simulink model "Mdl_BianchiOL_BladeB_WindFiltered"  (R2023a)
settings: Solver=FixedStepAuto  StartTime=0.0  StopTime=10.0  FixedStep=DT  RelTol=1e-3
values from neighbouring files (symbols this model uses):
  beta = 0.0 0.0017453292519943296 0.0034906585039886592 0.005235987755982989 0.0069813170079773184 0.0087266462599716477 0.010471975511965978 0.012217304763960306 0.013962634015954637 0.015707963267948967 0.017453292519943295 0.019198621771937627 0.020943951023931956 0.022689280275926284 0.024434609527920613 0.026179938779914941 0.027925268031909273 0.029670597283903605 0.031415926535897934 0.033161255787    [DD_Mdl1.sldd]
  Cq = 0.0 0.0 0.0 0.0 0.0 0.0 0.0 0.0 0.0 0.0 0.0 0.0 0.0 0.0 0.0 0.0 0.0 0.0 0.0 0.0 0.0 0.0 0.0 0.0 0.0 0.0 0.0 0.0 0.0 0.0 0.0 0.0 0.0 0.0 0.0 0.0 0.0 0.0 0.0 0.0 0.0 0.0 0.0 0.0 0.0 0.0 0.0 0.0 0.0 0.0 0.0 0.0 0.0 0.0 0.0 0.0 0.0 0.0 0.0 0.0 0.0 0.0 0.0 0.0 0.0 0.0 0.0 0.0 0.0 0.0 0.0 0.0 0.0 0.0 0.0 0.0 0.0 0.0 0.0 0.0 0.0 0.0 0.0 0.0 0.0 0.0 0.0 0.0 0.0 0.0 0.0 0.0 0.0 0.0 0.0 0.0 0.0 0.0 0.0 0.0    [DD_Mdl1.sldd]
  Ct = 0.0 0.0 0.0 0.0 0.0 0.0 0.0 0.0 0.0 0.0 0.0 0.0 0.0 0.0 0.0 0.0 0.0 0.0 0.0 0.0 0.0 0.0 0.0 0.0 0.0 0.0 0.0 0.0 0.0 0.0 0.0 0.0 0.0 0.0 0.0 0.0 0.0 0.0 0.0 0.0 0.0 0.0 0.0 0.0 0.0 0.0 0.0 0.0 0.0 0.0 0.0 0.0 0.0 0.0 0.0 0.0 0.0 0.0 0.0 0.0 0.0 0.0 0.0 0.0 0.0 0.0 0.0 0.0 0.0 0.0 0.0 0.0 0.0 0.0 0.0 0.0 0.0 0.0 0.0 0.0 0.0 0.0 0.0 0.0 0.0 0.0 0.0 0.0 0.0 0.0 0.0 0.0 0.0 0.0 0.0 0.0 0.0 0.0 0.0 0.0    [DD_Mdl1.sldd]
  lambda = 0.0 0.1 0.2 0.30000000000000004 0.4 0.5 0.60000000000000009 0.70000000000000007 0.8 0.9 1.0 1.1 1.2000000000000002 1.3 1.4000000000000001 1.5 1.6 1.7000000000000002 1.8 1.9000000000000001 2.0 2.1 2.2 2.3000000000000003 2.4000000000000004 2.5 2.6 2.7 2.8000000000000003 2.9000000000000004 3.0 3.1 3.2 3.3000000000000003 3.4000000000000004 3.5 3.6 3.7 3.8000000000000003 3.9000000000000004 4.0 4.100000    [DD_Mdl1.sldd]
  rho = 1.225    [DD_Mdl1.sldd]
  wecs = 3.0    [DD_Mdl1.sldd]    (also in wecsmatfile.m = struct)
libraries: Lib_WindFilter x1
Description:
  | Mdl2 (Mdl_BianchiOL_WindFiltered) with the blade model variant B (getBladeModelVersion B1/B2): WECS/BladeSchedule (bladeParamsMdl2) and WECS/LagrangeDyn instead of the constant matrix gains M\Q, M\K5, M\Ce
settings Model: DataDictionary=DD_Mdl1.sldd  Creator=ditt_aj  LastModifiedBy=jdi
settings SolverCC: AlgebraicLoopSolver=TrustRegion
settings DebuggingCC: UnconnectedInputMsg=warning  UnconnectedOutputMsg=warning  UnconnectedLineMsg=warning
settings ModelReferenceCC: EnableRefExpFcnMdlSchedulingChecks=on
settings SFSimCC: CustomCodeUndefinedFunction=UseInterfaceOnly
settings RTWCC: DLArmComputeVersion=19.05

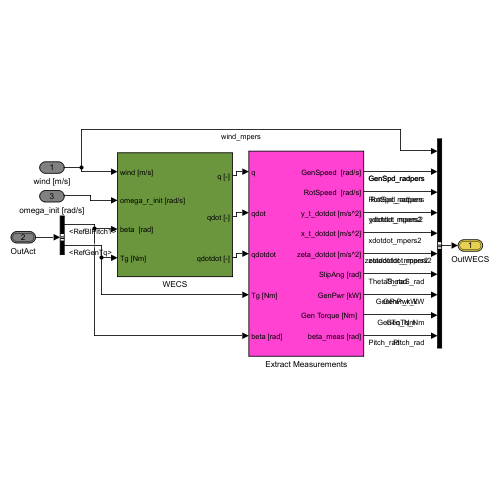
[thumbnail: Simulink's stored preview of the top-level diagram]
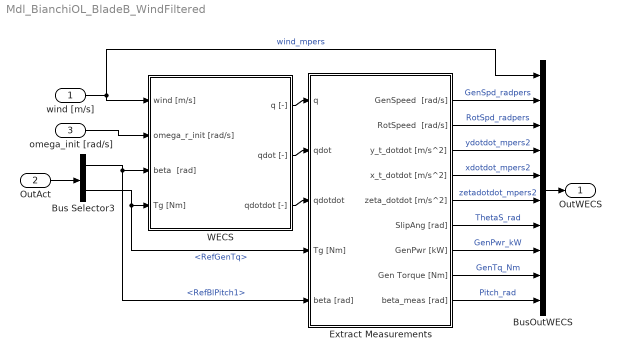
== system Mdl_BianchiOL_BladeB_WindFiltered ==
  wind [m/s] : Inport
  OutAct : Inport  Port=2  OutDataTypeStr=Bus: slBus2
  omega_init [rad/s] : Inport  Port=3
  Bus Selector3 : BusSelector  OutputSignals=RefBlPitch1,RefGenTq
  BusOutWECS : BusCreator  Inputs=10  OutDataTypeStr=Bus: slBus1
  Extract Measurements : Subsystem
  WECS : Subsystem
  OutWECS : Outport  OutDataTypeStr=Bus: slBus1
  wires:
  WECS/3(qdotdot [-]) -> Extract Measurements/3(qdotdot)
  omega_init [rad/s]/1 -> WECS/2(omega_r_init [rad/s])
  WECS/2(qdot [-]) -> Extract Measurements/2(qdot)
  WECS/1(q [-]) -> Extract Measurements/1(q)
  Extract Measurements/7(GenPwr [kW]) -> BusOutWECS/8  "GenPwr_kW"
  Extract Measurements/4(x_t_dotdot [m/s^2]) -> BusOutWECS/5  "xdotdot_mpers2"
  Extract Measurements/5(zeta_dotdot [m/s^2]) -> BusOutWECS/6  "zetadotdot_mpers2"
  Extract Measurements/6(SlipAng [rad]) -> BusOutWECS/7  "ThetaS_rad"
  Extract Measurements/9(beta_meas [rad]) -> BusOutWECS/10  "Pitch_rad"
  Extract Measurements/8("Gen Torque [Nm]  ") -> BusOutWECS/9  "GenTq_Nm"
  Extract Measurements/2(RotSpeed  [rad/s]) -> BusOutWECS/3  "RotSpd_radpers"
  Extract Measurements/3(y_t_dotdot [m/s^2]) -> BusOutWECS/4  "ydotdot_mpers2"
  BusOutWECS/1 -> OutWECS/1
  wind [m/s]/1 -> BusOutWECS/1, WECS/1(wind [m/s])  "wind_mpers"
  Extract Measurements/1(GenSpeed  [rad/s]) -> BusOutWECS/2  "GenSpd_radpers"
  OutAct/1 -> Bus Selector3/1
  Bus Selector3/2 -> Extract Measurements/4(Tg [Nm]), WECS/4(Tg [Nm])  "<RefGenTq>"
  Bus Selector3/1 -> Extract Measurements/5(beta [rad]), WECS/3(beta  [rad])  "<RefBlPitch1>"

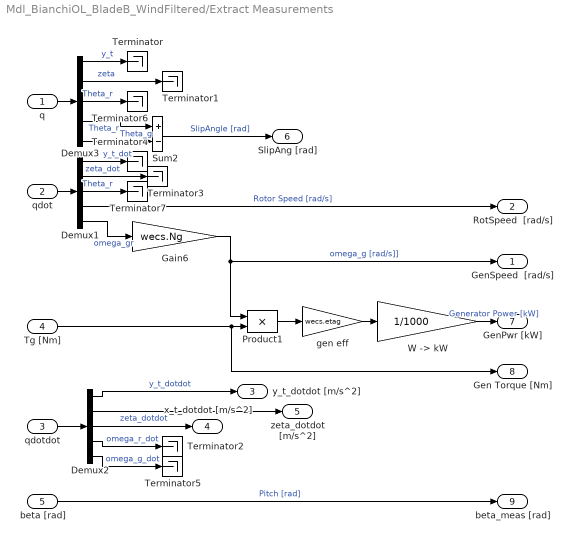
== system Mdl_BianchiOL_BladeB_WindFiltered/Extract Measurements ==
  q : Inport
  qdot : Inport  Port=2
  qdotdot : Inport  Port=3
  Tg [Nm] : Inport  Port=4
  beta [rad] : Inport  Port=5
  Demux1 : Demux  Outputs=5
  Demux2 : Demux  Outputs=5
  Demux3 : Demux  Outputs=5
  Gain6 : Gain  Gain=wecs.Ng
  Product1 : Product  RndMeth=Zero
  Sum2 : Sum  Inputs=+-
  Terminator{,1..7} (8 alike) : Terminator
  "W -> kW" : Gain  Gain=1/1000
  gen eff : Gain  Gain=wecs.etag
  GenSpeed  [rad/s] : Outport  VectorParamsAs1DForOutWhenUnconnected=off
  RotSpeed  [rad/s] : Outport  Port=2  VectorParamsAs1DForOutWhenUnconnected=off
  y_t_dotdot [m/s^2] : Outport  Port=3  VectorParamsAs1DForOutWhenUnconnected=off
  x_t_dotdot [m/s^2] : Outport  Port=4  VectorParamsAs1DForOutWhenUnconnected=off
  zeta_dotdot [m/s^2] : Outport  Port=5  VectorParamsAs1DForOutWhenUnconnected=off
  SlipAng [rad] : Outport  Port=6  VectorParamsAs1DForOutWhenUnconnected=off
  GenPwr [kW] : Outport  Port=7  VectorParamsAs1DForOutWhenUnconnected=off
  "Gen Torque [Nm]  " : Outport  Port=8  VectorParamsAs1DForOutWhenUnconnected=off
  beta_meas [rad] : Outport  Port=9  VectorParamsAs1DForOutWhenUnconnected=off
  wires:
  Demux1/2 -> Terminator3/1  "zeta_dot"
  Demux2/1 -> y_t_dotdot [m/s^2]/1  "y_t_dotdot"
  Gain6/1 -> GenSpeed  [rad/s]/1, Product1/1  "omega_g [rad/s]]"
  Demux1/1 -> Terminator4/1  "y_t_dot"
  qdot/1 -> Demux1/1
  Demux3/4 -> Sum2/1  "Theta_r"
  Demux3/5 -> Sum2/2  "Theta_g"
  Demux2/5 -> Terminator5/1  "omega_g_dot"
  Tg [Nm]/1 -> Product1/2, "Gen Torque [Nm]  "/1
  Demux2/4 -> Terminator2/1  "omega_r_dot"
  Sum2/1 -> SlipAng [rad]/1  "SlipAngle [rad]"
  Demux1/5 -> Gain6/1  "omega_gr"
  Product1/1 -> gen eff/1
  Demux3/2 -> Terminator1/1  "zeta"
  Demux2/2 -> zeta_dotdot [m/s^2]/1  "zeta_dotdot"
  Demux3/1 -> Terminator/1  "y_t"
  gen eff/1 -> "W -> kW"/1
  "W -> kW"/1 -> GenPwr [kW]/1  "Generator Power [kW]"
  q/1 -> Demux3/1
  qdotdot/1 -> Demux2/1
  Demux1/4 -> RotSpeed  [rad/s]/1  "Rotor Speed [rad/s]"
  beta [rad]/1 -> beta_meas [rad]/1  "Pitch [rad]"
  Demux2/3 -> x_t_dotdot [m/s^2]/1
  Demux3/3 -> Terminator6/1  "Theta_r"
  Demux1/3 -> Terminator7/1  "Theta_r"

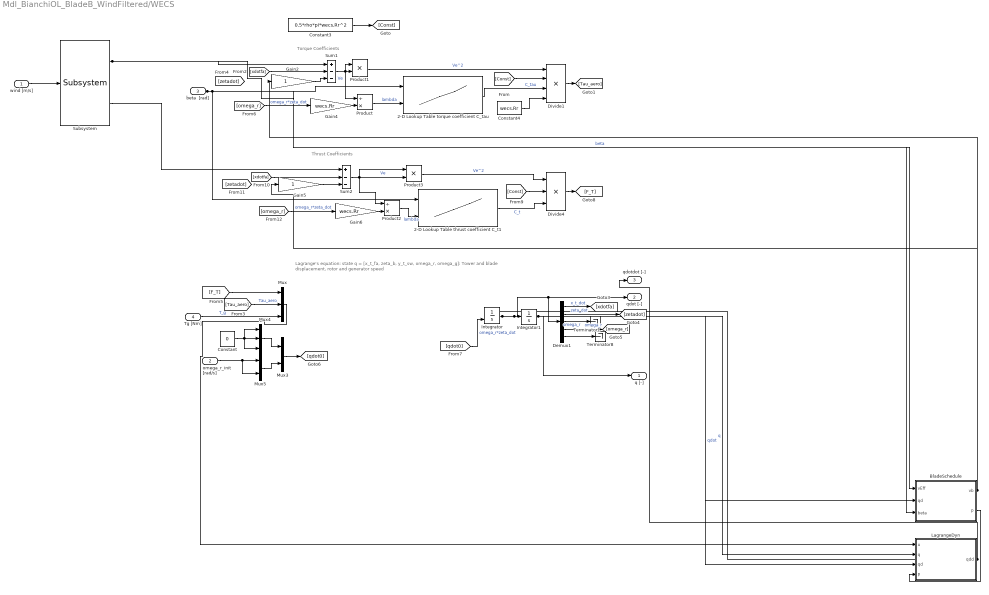
== system Mdl_BianchiOL_BladeB_WindFiltered/WECS ==
  note: Torque Coefficients
  note: Lagrange's equation: state q = [x_t_fa, zeta_b, y_t_sw, omega_r, omega_g]:
      | Tower and blade displacement, rotor and generator speed
  note: Thrust Coefficients
  wind [m/s] : Inport
  omega_r_init [rad/s] : Inport  Port=2
  beta  [rad] : Inport  Port=3
  Tg [Nm] : Inport  Port=4
  2-D Lookup Table thrust coefficient C_t1 : Lookup_n-D  BreakpointsForDimension1=beta  BreakpointsForDimension2=lambda  Table=Ct  InterpMethod=Cubic spline  InternalRulePriority=Speed  RndMeth=Simplest
      settings: InputPortMap=u0,u1
  2-D Lookup Table torque coefficient C_tau : Lookup_n-D  BreakpointsForDimension1=beta  BreakpointsForDimension2=lambda  Table=Cq  InterpMethod=Cubic spline  InternalRulePriority=Speed  RndMeth=Simplest
      settings: InputPortMap=u0,u1
  BladeSchedule : MATLAB Function  TreatAsAtomicUnit=on
  Constant : Constant  Value=0
  Constant3 : Constant  Value=0.5*rho*pi*wecs.Rr^2
  Constant4 : Constant  Value=wecs.Rr
  Demux1 : Demux  Outputs=5
  Divide1 : Product  Inputs=****
  Divide4 : Product  Inputs=***
  Gain2 : Gain
  Gain4 : Gain  Gain=wecs.Rr
  Gain5 : Gain
  Gain6 : Gain  Gain=wecs.Rr
  Integrator : Integrator  InitialConditionSource=external  InitialCondition=[0,0,0.75, 0.75]
  Integrator1 : Integrator  InitialCondition=[0,0,0,0,0]
  LagrangeDyn : MATLAB Function  TreatAsAtomicUnit=on
  Mux : Mux  Inputs=3
  Mux3 : Mux  Inputs=2
  Mux4 : Mux  Inputs=3
  Mux5 : Mux  Inputs=2
  Product : Product  Inputs=/*
  Product1 : Product  Inputs=**
  Product2 : Product  Inputs=/*
  Product3 : Product  Inputs=**
  Subsystem : Lib_WindFilter/Subsystem  SystemSampleTime=-1  VariantActivationTime=update diagram  Latency=0  AutoFrameSizeCalculation=off
  Sum1 : Sum  Inputs=+--
  Sum2 : Sum  Inputs=+--
  Terminator1 : Terminator
  Terminator8 : Terminator
  q [-] : Outport  VectorParamsAs1DForOutWhenUnconnected=off
  qdot [-] : Outport  Port=2  VectorParamsAs1DForOutWhenUnconnected=off
  qdotdot [-] : Outport  Port=3  VectorParamsAs1DForOutWhenUnconnected=off
  wires:
  Constant4/1 -> Divide1/4
  Sum1/1 -> Product/1, Product1/1, Product1/2  "Ve"
  Gain4/1 -> Product/2
  Divide1/1 -> [Tau_aero]
  [Const] -> Divide1/2
  2-D Lookup Table torque coefficient C_tau/1 -> Divide1/3  "C_tau"
  Integrator1/1 -> q [-]/1, LagrangeDyn/2(q)  "q"
  [F_T] -> Mux/1
  beta  [rad]/1 -> 2-D Lookup Table torque coefficient C_tau/1, 2-D Lookup Table thrust coefficient C_t1/1, BladeSchedule/3(beta)  "beta"
  Product/1 -> 2-D Lookup Table torque coefficient C_tau/2  "lambda"
  Product1/1 -> Divide1/1  "Ve^2"
  Integrator/1 -> Integrator1/1, Demux1/1, qdot [-]/1, BladeSchedule/2(qd), LagrangeDyn/3(qd)  "qdot"
  Constant3/1 -> [Const]
  [Tau_aero] -> Mux/2  "Tau_aero"
  Mux4/1 -> Mux3/1
  Constant/1 -> Mux4/3, Mux4/1, Mux4/2
  Mux5/1 -> Mux3/2
  Tg [Nm]/1 -> Mux/3  "T_g"
  Demux1/3 -> Terminator1/1  "omega_r"
  Demux1/5 -> Terminator8/1
  Demux1/1 -> [xdotfa]  "x_t_dot"
  [xdotfa] -> Sum1/2
  Demux1/2 -> [zetadot]  "zeta_dot"
  Demux1/4 -> [omega_r]  "omega_r"
  [omega_r] -> Gain4/1  "omega_r*zeta_dot"
  Gain2/1 -> Sum1/3
  omega_r_init [rad/s]/1 -> Mux5/2, Mux5/1
  Mux3/1 -> [qdot0]
  [qdot0] -> Integrator/2  "omega_r*zeta_dot"
  Gain5/1 -> Sum2/3
  [Const] -> Divide4/2
  Divide4/1 -> [F_T]
  [omega_r] -> Gain6/1  "omega_r*zeta_dot"
  Product3/1 -> Divide4/1  "Ve^2"
  Product2/1 -> 2-D Lookup Table thrust coefficient C_t1/2  "lambda"
  [xdotfa] -> Sum2/2
  Sum2/1 -> Product2/1, Product3/1, Product3/2  "Ve"
  Gain6/1 -> Product2/2
  2-D Lookup Table thrust coefficient C_t1/1 -> Divide4/3  "C_t"
  Subsystem/2 -> Sum2/1
  Subsystem/1 -> Sum1/1, BladeSchedule/1(vEff)
  wind [m/s]/1 -> Subsystem/1
  BladeSchedule/1(vb) -> Gain2/1, Gain5/1
  Mux/1 -> LagrangeDyn/1(u)
  BladeSchedule/2(p) -> LagrangeDyn/4(p)
  LagrangeDyn/1(qdd) -> Integrator/1, qdotdot [-]/1

== matlab function Mdl_BianchiOL_BladeB_WindFiltered/WECS/LagrangeDyn ==
  data: u input; qdd output; q input; qd input; p input; wecs parameter
function qdd = LagrangeDyn(u, q, qd, p, wecs)
% Lagrange model (initModel5MWNREL) with blade parameters p = [rr; rb; Kb; mb]
rr = p(1); rb = p(2); Kb = p(3); mb = p(4); N = wecs.N;
Bb = 2*wecs.zetab*sqrt(Kb*mb);
cSw = 3/(2*wecs.H);
M = [wecs.mt + N*mb, N*mb*rr, 0, 0, 0; N*mb*rr, N*mb*rr^2, 0, 0, 0; 0, 0, wecs.mt, 0, 0; 0, 0, 0, wecs.JrL, 0; 0, 0, 0, 0, wecs.Jg*wecs.Ng^2];
Ce = [wecs.Bt, 0, 0, 0, 0; 0, N*Bb*rr^2, 0, 0, 0; 0, 0, wecs.Btsw, 0, 0; 0, 0, 0, wecs.Bs, -wecs.Bs; 0, 0, 0, -wecs.Bs, wecs.Bs];
K5 = [wecs.Kt, 0, 0, 0, 0; 0, N*Kb*rr^2, 0, 0, 0; 0, 0, wecs.Ktsw, 0, 0; 0, 0, 0, wecs.Ks, -wecs.Ks; 0, 0, 0, -wecs.Ks, wecs.Ks];
Q3 = [1, 0, 0; rb, 0, 0; 0, -cSw*(1 - wecs.cMx), -cSw*wecs.cMx*wecs.Ng; 0, 1, 0; 0, 0, -wecs.Ng];
qdd = M \ (Q3*u(:) - K5*q(:) - Ce*qd(:));

== matlab function Mdl_BianchiOL_BladeB_WindFiltered/WECS/BladeSchedule ==
  data: vEff input; vb output; qd input; beta input; p output; wecs parameter
function [vb, p] = BladeSchedule(vEff, qd, beta, wecs)
% Blade model variant B (bladeParamsMdl2, parameters wecs.blade* of
% initModel5MWNREL): modal mass mb at the radius rr, thrust load point rb and
% stiffness Kb at the tip speed ratio lambda0 (without the blade velocity)
% and the pitch angle; vb: velocity of the load point (relative wind)
lam0 = wecs.Rr*qd(4)/max(vEff - qd(1), 0.5);
[rr, rb, Kb, mb] = bladeParamsMdl2(wecs, lam0, beta(1), 0);
vb = rb*qd(2);
p = [rr; rb; Kb; mb];
